simulink subsystem "PhaseShift"  (R2026a)
settings: Solver=VariableStepAuto
undefined symbols (not defined in the file): Filter_Current_FilterTimeConst, Filter_Current_SensorTimeConst, FOC, FOC_LUT_ParkClake_AtanLut
settings Model: Creator=kara  LastModifiedBy=Cheng

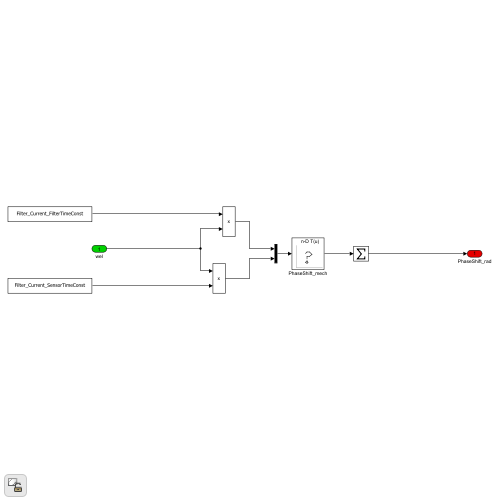
[thumbnail: Simulink's stored preview of the top-level diagram]
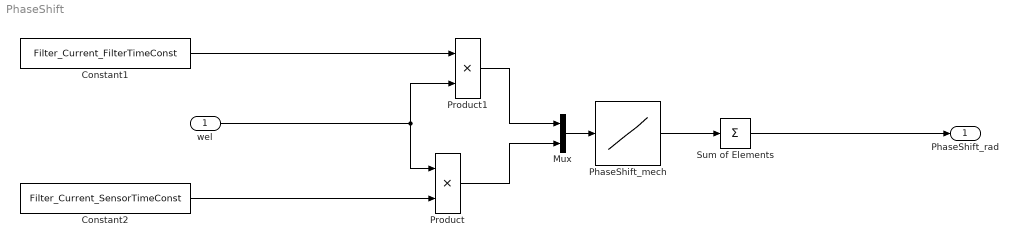
== system PhaseShift ==
  wel : Inport
  Constant1 : Constant  Value=Filter_Current_FilterTimeConst  SampleTime=-1
  Constant2 : Constant  Value=Filter_Current_SensorTimeConst  SampleTime=-1
  Mux : Mux  Inputs=2
  PhaseShift_mech : Lookup_n-D  NumberOfTableDimensions=1  BreakpointsForDimension1=FOC.LUT.ParkClake.AtanxValue  Table=FOC_LUT_ParkClake_AtanLut  InternalRulePriority=Speed  RndMeth=Simplest
  Product : Product  OutDataTypeStr=SIScaling
  Product1 : Product  OutDataTypeStr=SIScaling
  Sum of Elements : Sum  Inputs=+
  PhaseShift_rad : Outport
  wires:
  wel/1 -> Product1/2, Product/1
  Product1/1 -> Mux/1
  Product/1 -> Mux/2
  Mux/1 -> PhaseShift_mech/1
  PhaseShift_mech/1 -> Sum of Elements/1
  Sum of Elements/1 -> PhaseShift_rad/1
  Constant1/1 -> Product1/1
  Constant2/1 -> Product/2
